simulink model "BEV_system_model"  (R2026a)
settings: Solver=daessc  StartTime=0  StopTime=100  MaxStep=0.1  AbsTol=1e-3  EnableMultiTasking=on
PreLoadFcn:
  | defineBus_HighVoltage
  | defineBus_Rotational
PostLoadFcn:
  | BEV_setup
libraries: nesl_utility x2
Description:
  | Battery Electric Vehicle drive cycle simulation
settings Model: FPTRunName=Active  Creator=MathWorks  LastModifiedBy=ythvg
settings SolverCC: MinimalZcImpactIntegration=on
settings DataIOCC: MaxDataPoints=15000
settings DebuggingCC: UnderspecifiedInitializationDetection=Classic  UnitsInconsistencyMsg=none
settings HardwareCC: ProdHWDeviceType=32-bit Generic
settings GRTTargetCC: CombineOutputUpdateFcns=off  GRTInterface=on
settings ConfigComp: CovScope=Subsystem  CovPath=Driver & Environment/Torque Limiter  CovMetricSettings=dcmw
settings SimscapeCC: SimscapeNominalValues="[{\"value\":\"20\",\"unit\":\"A\"},{\"value\":\"1\",\"unit\":\"bar\"},{\"value\":\"1\",\"unit\":\"cm^2\"},{\"value\":\"1\",\"unit\":\"cm^3/s\"},{\"value\":\"1\",\"unit\":\"kJ/kg\"},{\"value\":\"1\",\"unit\":\"kW\"},{\"value\":\"1\",\"unit\":\"l\"},{\"value\":\"1\",\"unit\":\"N\"},{\"value\":\"40\",\"unit\":\"N*m\"},{\"value\":\"350\",\"unit\":\"V\"}]"  SimscapeLogSimulationStatistics=on  SimscapeLogName=logoutssc  SimscapeLogLimitData=off

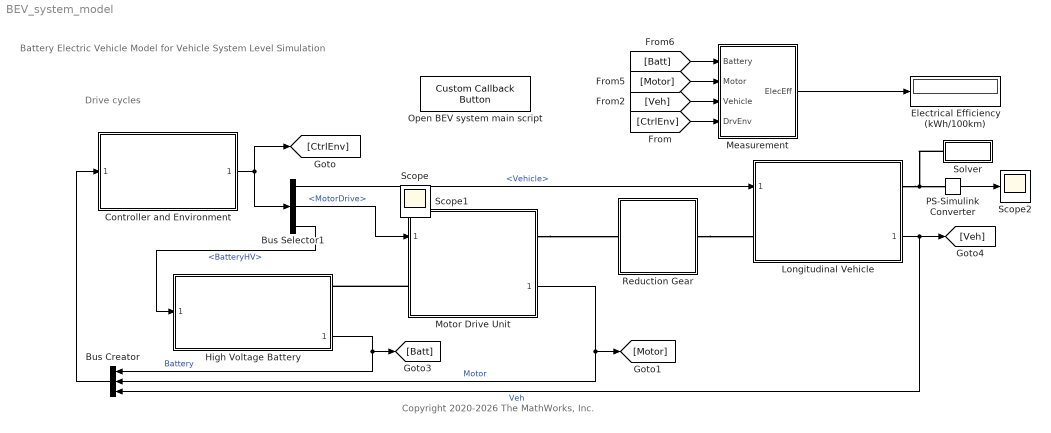
== system BEV_system_model ==
  note: Drive cycles
  note: Battery Electric Vehicle Model for Vehicle System Level Simulation
  note: Copyright 2020-2026 The MathWorks, Inc.
  Bus Creator : BusCreator  Inputs=3
  Bus Selector1 : BusSelector  OutputSignals=Vehicle,MotorDrive,BatteryHV
  Controller and Environment : Subsystem  ReferencedSubsystem=CtrlEnv_Basic_refsub
      settings: OpenFcn=|
      | % Look under mask:
      | open_system(gcb, "force")
  Electrical Efficiency (kWh/100km) : Display
  High Voltage Battery : Subsystem  ReferencedSubsystem=BatteryHV_Basic_refsub
      settings: PortSchema="{\"entries\":[{\"content\":{\"sides\":[{\"content\":{\"connectorIds\":[\"In1\"]},\"type\":\"ConnectorPlacement.EquallySpacedRectSide\",\"uuid\":\"5db791d4-e733-413a-9b9b-d79e76ac9bb0\"},{\"content\":{\"connectorIds\":[\"RConn1\",\"RConn2\",\"Out1\"],\"side\":\"RIGHT\"},\"type\":\"ConnectorPlacement.EquallySpacedRectSide\",\"uuid\":\"0c12beb5-1dc0-4de1-849a-92aaa1061486\"},{\"content\":{\"side\":\"TOP\"},\"type\":\"ConnectorPlacement.EquallySpacedRectSide\",\"uuid\":\"758dbf8c-c8ee-4b73-af05-227531b6198b\"},{\"content\":{\"side\":\"HIDDEN\"},\"type\":\"ConnectorPlacement.EquallySpacedRectSide\",\"uuid\":\"fa4920b8-ec2a-4218-a476-41d1e0d36381\"}]},\"type\":\"ConnectorPlacement.EquallySpacedConnector\",\"uuid\":\"d828a3e3-8826-44df-b770-75b0ad7bf91b\"}],\"packageUris\":[\"http://schema.mathworks.com/mf0/Connector/R2020b\"],\"version\":\"1.0\"}"
      settings: OpenFcn=|
      | % Look under mask:
      | open_system(gcb, "force")
  Longitudinal Vehicle : Subsystem  ReferencedSubsystem=Vehicle1D_Basic_refsub
      settings: PortSchema="{\"entries\":[{\"content\":{\"sides\":[{\"content\":{\"connectorIds\":[\"In1\",\"LConn1\"]},\"type\":\"ConnectorPlacement.EquallySpacedRectSide\",\"uuid\":\"1278221b-4210-4fc4-9018-d7f4555b8d65\"},{\"content\":{\"connectorIds\":[\"RConn1\",\"Out1\"],\"side\":\"RIGHT\"},\"type\":\"ConnectorPlacement.EquallySpacedRectSide\",\"uuid\":\"ae02a7d1-22cf-4294-9907-02c3616e735c\"},{\"content\":{\"side\":\"TOP\"},\"type\":\"ConnectorPlacement.EquallySpacedRectSide\",\"uuid\":\"498bee53-b001-4331-968a-8dad39da1579\"}]},\"type\":\"ConnectorPlacement.EquallySpacedConnector\",\"uuid\":\"c28a1585-5582-45c2-8974-ffffcb6069ab\"}],\"packageUris\":[\"http://schema.mathworks.com/mf0/Connector/R2020b\"],\"version\":\"1.0\"}"
      settings: OpenFcn=|
      | % Look under mask:
      | open_system(gcb, "force")
  Measurement : Subsystem
  Motor Drive Unit : Subsystem  ReferencedSubsystem=MotorDriveUnit_Basic_refsub
      settings: PortSchema="{\"entries\":[{\"content\":{\"sides\":[{\"content\":{\"connectorIds\":[\"In1\",\"LConn1\"]},\"type\":\"ConnectorPlacement.EquallySpacedRectSide\",\"uuid\":\"67ecf7a6-5e47-4eb7-8bef-e90b74b30c45\"},{\"content\":{\"connectorIds\":[\"RConn1\",\"Out1\"],\"side\":\"RIGHT\"},\"type\":\"ConnectorPlacement.EquallySpacedRectSide\",\"uuid\":\"a9028cc8-cfc1-431e-b7d7-768ed50af379\"},{\"content\":{\"side\":\"TOP\"},\"type\":\"ConnectorPlacement.EquallySpacedRectSide\",\"uuid\":\"a0687387-3123-4d08-86fe-456eeb37040f\"}]},\"type\":\"ConnectorPlacement.EquallySpacedConnector\",\"uuid\":\"6bbfd8f6-f8bb-42c4-a351-7db31f6b96f0\"}],\"packageUris\":[\"http://schema.mathworks.com/mf0/Connector/R2020b\"],\"version\":\"1.0\"}"
      settings: OpenFcn=|
      | % Look under mask:
      | open_system(gcb, "force")
  Open BEV system main script : CustomCallbackButton  Configuration="{\"components\":[{\"name\":\"BackgroundImageComponent\",\"settings\":{\"image\":{\"size\":[0,0],\"src\":\"default\",\"srcOrientation\":\"Right\"},\"position\":[0,0,1,1]}},{\"name\":\"ButtonStateComponent\",\"settings\":{\"buttonType\":\"momentary\",\"clickFcn\":\"edit(\\\"BEV_main_script\\\")\",\"onValue\":1,\"position\":[0,0,1,1],\"pressDelay\":\"500\",\"pressFcn\":\"\",\"repeatInterval\":\"0\",\"states\":[{\"horizontalAlignment\":\"center\",\"image\":{\"position\":[0,0,1,1],\"size\":[1,1],\"src\":\"default\",\"srcOrientation\":\"Right\"},\"label\":{\"color\":[0.01176470588,0.01176470588,0.01176470588,1],\"icon\":{\"size\":[0,0],\"src\":\"default\",\"srcOrientation\":\"Right\"},\"iconOffset\":0,\"iconPlacement\":\"left\",\"opacity\":1,\"show\":true,\"text\":{\"content\":\"Open script\",\"font\":\"Helvetica\"}},\"labelOffset\":[0,0],\"verticalAlignment\":\"middle\"},{\"horizontalAlignment\":\"center\",\"image\":{\"position\":[0,0,1,1],\"size\":[1,1],\"src\":\"default\",\"srcOrientation\":\"Right\"},\"label\":{\"color\":[0.01176470588,0.01176470588,0.01176470588,1],\"icon\":{\"size\":[0,0],\"src\":\"default\",\"srcOrientation\":\"Right\"},\"iconOffset\":0,\"iconPlacement\":\"left\",\"opacity\":1,\"show\":true,\"text\":{\"content\":\"Open script\",\"font\":\"Helvetica\"}},\"labelOffset\":[0,0],\"verticalAlignment\":\"middle\"},{\"horizontalAlignment\":\"center\",\"image\":{\"position\":[0,0,1,1],\"size\":[1,1],\"src\":\"default\",\"srcOrientation\":\"Right\"},\"label\":{\"color\":[0.01176470588,0.01176470588,0.01176470588,1],\"icon\":{\"size\":[0,0],\"src\":\"default\",\"srcOrientation\":\"Right\"},\"iconOffset\":0,\"iconPlacement\":\"left\",\"opacity\":1,\"show\":true,\"text\":{\"content\":\"Open script\",\"font\":\"Helvetica\"}},\"labelOffset\":[0,0],\"verticalAlignment\":\"middle\"},{\"horizontalAlignment\":\"center\",\"image\":{\"position\":[0,0,1,1],\"size\":[1,1],\"src\":\"default\",\"srcOrientation\":\"Right\"},\"label\":{\"color\":[0.01176470588,0.01176470588,0.01176470588,1],\"icon\":{\"size\":[0,0],\"src\":\"default\",\"srcOrientation\":\"Right\"},\"iconOffset\":0,\"iconPlacement\":\"left\",\"opacity\":1,\"show\":true,\"text\":{\"content\":\"Open script\",\"font\":\"Helvetica\"}},\"labelOffset\":[0,0],\"verticalAlignment\":\"middle\"}]}},{\"name\":\"ForegroundImageComponent\",\"settings\":{\"image\":{\"size\":[0,0],\"src\":\"default\",\"srcOrientation\":\"Right\"},\"isForeground\":1,\"position\":[0,0,1,1]}}],\"derived\":{\"blockParameters\":{\"AutoActivate\":true,\"ButtonText\":\"Open script\",\"ButtonType\":\"Momentary\",\"ClickFcn\":\"edit(\\\"BEV_main_script\\\")\",\"OnValue\":1,\"PressDelay\":\"500\",\"PressFcn\":\"\",\"RepeatInterval\":\"0\",\"fixedAspectRatio\":\"off\"}},\"settings\":{\"BindingType\":\"standalone\",\"autoActivate\":true,\"backgroundColor\":[244,244,244,1],\"backgroundOffset\":0.2,\"backgroundOpacity\":1,\"fixedAspectRatio\":\"off\",\"foregroundColor\":[0.01176470588,0.01176470588,0.01176470588,1],\"migratedFromLegacy\":true,\"useBackgroundColor\":true,\"variant\":\"callback\",\"version\":\"R2025a\"},\"type\":\"Button\"}"  CustomBackgroundColor="{\"color\":[0.9568627451,0.9568627451,0.9568627451],\"show\":true}"
  PS-Simulink Converter : nesl_utility/PS-Simulink Converter  PhysicalDomain=network_engine_domain  SubClassName=ps_output  LeftPortType=input  RightPortType=output  PseudoPeriodic=off  Frequencies=[]  VectorFormat=inherit  Unit=m/s  AffineConversion=off
  Reduction Gear : Subsystem  ReferencedSubsystem=Reducer_Basic_refsub
      settings: OpenFcn=|
      | % Look under mask:
      | open_system(gcb, "force")
  Scope2 : Scope
  Solver : Subsystem
  Scope : Scope
      settings: ActiveDisplayYMinimum=-1.01075  ActiveDisplayYMaximum=0.74923
  Scope1 : Scope
      settings: ActiveDisplayYMinimum=-0.10303  ActiveDisplayYMaximum=0.07637  DataLoggingVariableName=ScopeData2
  wires:
  [Veh] -> Measurement/3(Vehicle)
  [Motor] -> Measurement/2(Motor)
  [Batt] -> Measurement/1(Battery)
  High Voltage Battery/1 -> [Batt], Bus Creator/1  "Battery"
  Longitudinal Vehicle/1 -> [Veh], Bus Creator/3  "Veh"
  [CtrlEnv] -> Measurement/4(DrvEnv)
  Bus Selector1/2 -> Motor Drive Unit/1  "<MotorDrive>"
  Motor Drive Unit/1 -> Bus Creator/2, [Motor]  "Motor"
  Bus Creator/1 -> Controller and Environment/1
  Bus Selector1/3 -> High Voltage Battery/1  "<BatteryHV>"
  Bus Selector1/1 -> Longitudinal Vehicle/1  "<Vehicle>"
  Measurement/1(ElecEff) -> Electrical Efficiency (kWh/100km)/1
  Controller and Environment/1 -> [CtrlEnv], Bus Selector1/1
  PS-Simulink Converter/1 -> Scope2/1
  connections:
  Motor Drive Unit/LConn1 -- High Voltage Battery/RConn1
  Reduction Gear/RConn1 -- Longitudinal Vehicle/LConn1
  Motor Drive Unit/RConn1 -- Reduction Gear/LConn1
  Longitudinal Vehicle/RConn1 -- Solver/LConn1 -- PS-Simulink Converter/LConn1

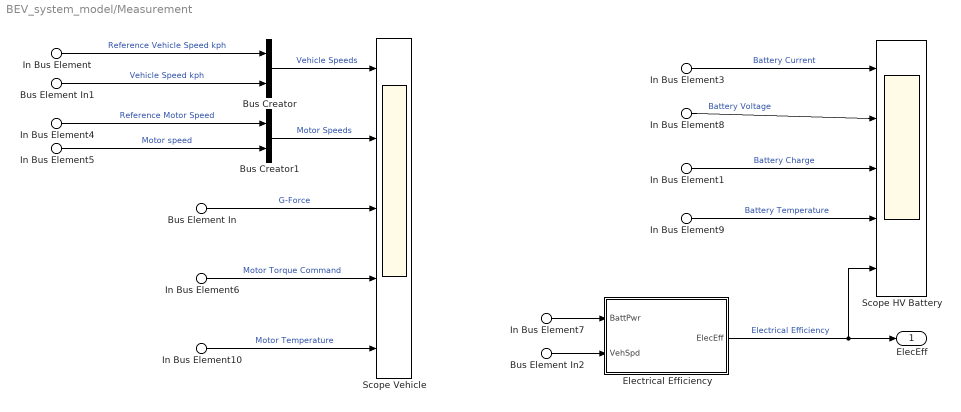
== system BEV_system_model/Measurement ==
  In Bus Element3 : Inport  PortName=Battery  Element=Current
  In Bus Element1 : Inport  PortName=Battery  Element=Charge
  In Bus Element7 : Inport  PortName=Battery  Element=Power
  In Bus Element9 : Inport  PortName=Battery  Element=Temp
  In Bus Element8 : Inport  PortName=Battery  Element=Voltage
  In Bus Element6 : Inport  Port=2  PortName=Motor  Element=TrqCmd
  In Bus Element5 : Inport  Port=2  PortName=Motor  Element=MotorSpd
  In Bus Element10 : Inport  Port=2  PortName=Motor  Element=MotorTemp
  Bus Element In : Inport  Port=3  PortName=Vehicle  Element=G
  Bus Element In2 : Inport  Port=3  PortName=Vehicle  Element=VehSpdKph
  Bus Element In1 : Inport  Port=3  PortName=Vehicle  Element=VehSpdKph
  In Bus Element : Inport  Port=4  PortName=DrvEnv  Element=Info.VehSpdRef
  In Bus Element4 : Inport  Port=4  PortName=DrvEnv  Element=Info.MotorSpdRef
  Bus Creator : BusCreator  Inputs=2
  Bus Creator1 : BusCreator  Inputs=2
  Electrical Efficiency : Subsystem
  Scope HV Battery : Scope  NumInputPorts=5
      settings: ActiveDisplayYMinimum=-200.18489790740119  ActiveDisplayYMaximum=229.08664516453314
  Scope Vehicle : Scope  NumInputPorts=5
      settings: ActiveDisplayYMinimum=-817.66255630430646  ActiveDisplayYMaximum=7289.6405451631408  DataLoggingVariableName=ScopeData2
  ElecEff : Outport
  wires:
  In Bus Element1/1 -> Scope HV Battery/3  "Battery Charge"
  In Bus Element3/1 -> Scope HV Battery/1  "Battery Current"
  In Bus Element/1 -> Bus Creator/1  "Reference Vehicle Speed kph"
  Bus Element In1/1 -> Bus Creator/2  "Vehicle Speed kph"
  In Bus Element5/1 -> Bus Creator1/2  "Motor speed"
  In Bus Element4/1 -> Bus Creator1/1  "Reference Motor Speed"
  Bus Creator1/1 -> Scope Vehicle/2  "Motor Speeds"
  Bus Element In/1 -> Scope Vehicle/3  "G-Force"
  Bus Creator/1 -> Scope Vehicle/1  "Vehicle Speeds"
  In Bus Element6/1 -> Scope Vehicle/4  "Motor Torque Command"
  In Bus Element9/1 -> Scope HV Battery/4  "Battery Temperature"
  In Bus Element10/1 -> Scope Vehicle/5  "Motor Temperature"
  In Bus Element8/1 -> Scope HV Battery/2  "Battery Voltage"
  Electrical Efficiency/1(ElecEff) -> Scope HV Battery/5, ElecEff/1  "Electrical Efficiency"
  In Bus Element7/1 -> Electrical Efficiency/1(BattPwr)
  Bus Element In2/1 -> Electrical Efficiency/2(VehSpd)

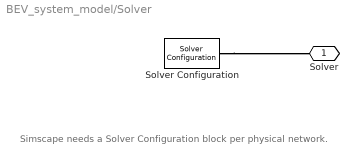
== system BEV_system_model/Solver ==
  note: Simscape needs a Solver Configuration block per physical network.
  Solver Configuration : nesl_utility/Solver Configuration  PhysicalDomain=network_engine_domain  SubClassName=solver  LeftPortType=input  RightPortType=generic  Tones=[]  Harmonics=[]  SimulateNoise=off  Profile=off  UseLocalSampling=off  EnableSwitchedLinearOptims=on  FrequencyDomain=off  UseCCode=off  RelTol=0.001  AbsTol=1e-06  MinStep=1e-09  ToWorkspace=off  RevertToSquareIcSolve=off  NumHomotopyIterations=100  PhasorMode=off  PhasorModeNumHarmonics=1  ConsistencySolver=NEWTON_FTOL  CanonicalOrdering=UNORDERED  OptimizeIntermediates=UNOPTIMIZED  IndexReductionMethod=DerivativeReplacement  DoDC=off  ResidualTolerance=1e-6  ConsistencyTolSource=GLOBAL  ConsistencyAbsTol=0.001  ConsistencyRelTol=0.001  ConsistencyTolFactor=0.001  UseLocalSolver=off  LocalSolverChoice=NE_BACKWARD_EULER_ADVANCER  ResolveIndetEquations=on  FunctionEvalNumThread=1  LocalSolverSampleTime=0.01  DoFixedCost=off  MaxNonlinIter=3  MaxModeIter=2  ComputeImpulses=off  ImpulseIterations=2  LinearAlgebra=auto  LinearAlgebraNumThread=0  EquationFormulation=NE_TIME_EF  DelaysMemoryBudget=1024  AutomaticFiltering=on  FilteringTimeConstant=0.001  PartitionStorageMethod=AS_NEEDED  PartitionMemoryBudget=1024  PartitionMethod=FAST  MultibodyUseLocalSolver=off  MultibodyLocalSolverChoice=ODE1  MultibodyLocalSolverSampleTime=0.001
      settings: AttributesFormatString=Local solver %<UseLocalSolver>
  Solver : PMIOPort  Side=Left
  connections:
  Solver Configuration/RConn1 -- Solver/RConn1

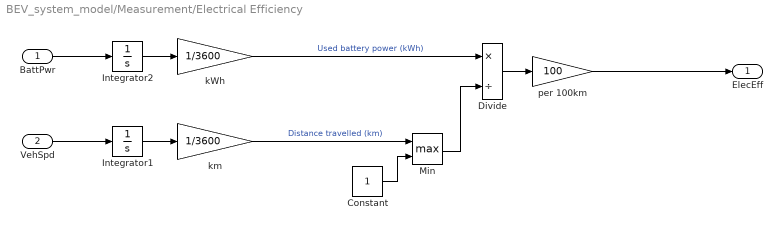
== system BEV_system_model/Measurement/Electrical Efficiency ==
  BattPwr : Inport  Unit=kW
  VehSpd : Inport  Port=2  Unit=km/hr
  Constant : Constant
  Divide : Product  Inputs=*/
  Integrator1 : Integrator
  Integrator2 : Integrator
  Min : MinMax  Function=max  Inputs=2
  kWh : Gain  Gain=1/3600
  km : Gain  Gain=1/3600
  per 100km : Gain  Gain=100
  ElecEff : Outport  Unit=kW*hr/(100*km)
  wires:
  km/1 -> Min/1  "Distance travelled (km)"
  Constant/1 -> Min/2
  Integrator2/1 -> kWh/1
  Divide/1 -> per 100km/1
  Integrator1/1 -> km/1
  Min/1 -> Divide/2
  kWh/1 -> Divide/1  "Used battery power (kWh)"
  per 100km/1 -> ElecEff/1
  BattPwr/1 -> Integrator2/1
  VehSpd/1 -> Integrator1/1
